simulink model "commhdlQPSKTxRxLoopback"  (R2025b)
settings: Solver=FixedStepDiscrete  StartTime=0.0  StopTime=stopTime  RelTol=1e-3
PostLoadFcn:
  | hScopeConfig = get_param([gcs '/Receiver/QPSK Rx/Frequency and Time Synchronizer/Symbol Synchronizer/No HDL/QPSK Receiver Eye Diagram'],'ScopeConfiguration');
  | 
  | hScopeConfig.OpenAtSimulationStart = false;
  | hScopeConfig.Visible = false;
  | SamplesPerSymbol = 4;
  | %UpsamplesRx = 1;
  | clear hScopeConfig
InitFcn:
  | commhdlQPSKTxRxModelInit;
  | % Rate bridge: ADRV9002/Jupiter radio runs at 15.36 MHz = 2x the 7.68 MHz
  | % (4 samples/symbol @ Rsym=1.92 MHz) the QPSK Rx requires. The deployed
  | % Receiver must downsample the ADC stream by 2. UpsamplesRx=1 fed the QPSK
  | % Rx 8 sps (2x-upsampled) and broke symbol sync / the loopback bit check.
  | UpsamplesRx = 1;   %% T8 RATE FIX: rail 15.36e6 == ADC bus rate,
  | %% no ingress decimation (was 2 when the rail sat on the 7.68e6 rung)
  | UpsamplesTx = 1;
  | clear simTimingOffset;
StopFcn:
  | if exist('simTimingOffset','var')
  |   disp('Simulation completed');
  |   %QPSKTxRxVerification;
  | end
undefined symbols (not defined in the file or in its folder): Add, Config, fsym, randsrc, RandStream, Rsym, Shift
libraries: hdlsllib x141, simulink x43, dspsigops x34, dsphdlfiltering2 x6, dsphdlsigops2 x4, dsphdlmathfun2 x4, commdigbbndpm3 x4, dspmlti4 x2, commchan3 x1, commrflib2 x1, commcnvcod2 x1
(part 6 of 8)

== system commhdlQPSKTxRxLoopback/TxRxComposite/Receiver/QPSK Rx/Frequency and Time Synchronizer/Preamble Detector/Peak Search ==
  note: peak picker
  corr : Inport
  thresholdExceeded : Inport  Port=2
  validIn : Inport  Port=3
  Compare To Constant : simulink/Logic and Bit Operations/Compare To Constant  relop===  const=samplesPerFrame1x - 1  OutDataTypeStr=boolean
  Logical Operator : Logic  IconShape=distinctive  AllPortsSameDT=off  OutDataTypeStr=boolean
  Logical Operator4 : Logic  IconShape=distinctive  AllPortsSameDT=off  OutDataTypeStr=boolean
  Relational Operator : RelationalOperator  Operator=>  OutDataTypeStr=boolean  InputSameDT=off
  Terminator : Terminator
  Unit Delay Enabled Synchronous : hdlsllib/Discrete/Unit Delay Enabled Synchronous  InitialCondition=0.0  SampleTime=-1
  Unit Delay Enabled Synchronous1 : hdlsllib/Discrete/Unit Delay Enabled Synchronous  InitialCondition=0.0  SampleTime=-1
  Unit Delay Enabled Resettable Synchronous : hdlsllib/Discrete/Unit Delay Enabled Resettable Synchronous  InitialCondition=0.0  SampleTime=-1
  Unit Delay Enabled Resettable Synchronous1 : hdlsllib/Discrete/Unit Delay Enabled Resettable Synchronous  InitialCondition=0.0  SampleTime=-1
  timing Reference : hdlsllib/Sources/HDL Counter  CountType=Count limited  CountInit=0  CountStep=1  CountMax=samplesPerFrame1x - 1  CountFromType=Initial value  CountFrom=0  CountResetPort=off  CountLoadPort=off  CountEnbPort=on  CountDirPort=off  CountHitOutputPort=off  CountDataType=Unsigned  CountWordLen=nextpow2(samplesPerFrame1x - 1)  CountFracLen=0  CountSampTime=1
  timing Reference Long : hdlsllib/Sources/HDL Counter  CountType=Free running  CountInit=0  CountStep=1  CountMax=samplesPerFrame1x - 1  CountFromType=Initial value  CountFrom=0  CountResetPort=off  CountLoadPort=off  CountEnbPort=on  CountDirPort=off  CountHitOutputPort=off  CountDataType=Unsigned  CountWordLen=32  CountFracLen=0  CountSampTime=1
  timingOffset : Outport
  done : Outport  Port=2
  success : Outport  Port=3
  p1c_tref : Outport  Port=4
  p1c_treflong : Outport  Port=5
  p1c_runmax : Outport  Port=6
  p1c_newpk : Outport  Port=7
  p1c_heldts : Outport  Port=8
  wires:
  Unit Delay Enabled Synchronous1/1 -> Terminator/1, p1c_heldts/1
  Unit Delay Enabled Synchronous/1 -> timingOffset/1
  Logical Operator4/1 -> Unit Delay Enabled Resettable Synchronous/2, Unit Delay Enabled Synchronous1/2, Unit Delay Enabled Synchronous/2, p1c_newpk/1
  Unit Delay Enabled Resettable Synchronous1/1 -> success/1
  Unit Delay Enabled Resettable Synchronous/1 -> Relational Operator/2, p1c_runmax/1
  Relational Operator/1 -> Logical Operator4/1
  Logical Operator/1 -> Unit Delay Enabled Resettable Synchronous/3, done/1, Unit Delay Enabled Resettable Synchronous1/3
  Compare To Constant/1 -> Logical Operator/2
  corr/1 -> Relational Operator/1, Unit Delay Enabled Resettable Synchronous/1
  thresholdExceeded/1 -> Logical Operator4/2, Unit Delay Enabled Resettable Synchronous1/1, Unit Delay Enabled Resettable Synchronous1/2
  timing Reference/1 -> Compare To Constant/1, Unit Delay Enabled Synchronous/1, p1c_tref/1
  timing Reference Long/1 -> Unit Delay Enabled Synchronous1/1, p1c_treflong/1
  validIn/1 -> timing Reference Long/1, timing Reference/1, Logical Operator/1

== system commhdlQPSKTxRxLoopback/TxRxComposite/Receiver/QPSK Rx/Frequency and Time Synchronizer/Preamble Detector/Timing Adjust ==
  timingOffset : Inport
  timingOffsetValid : Inport  Port=2
  dataIn : Inport  Port=3
  validIn : Inport  Port=4
  Delay{,1..4} (5 alike) : Delay  DelayLength=1
  Logical Operator : Logic  AllPortsSameDT=off  OutDataTypeStr=boolean
  Logical Operator1 : Logic  Operator=NOT  AllPortsSameDT=off  OutDataTypeStr=boolean
  Logical Operator2 : Logic  Inputs=3  AllPortsSameDT=off  OutDataTypeStr=boolean
  No HDL : Subsystem
  Relational Operator : RelationalOperator  Operator===  OutDataTypeStr=boolean  InputSameDT=off
  State Register : hdlsllib/Discrete/Unit Delay Enabled Resettable Synchronous  InitialCondition=0.0  SampleTime=-1
  Unit Delay Enabled Synchronous3 : hdlsllib/Discrete/Unit Delay Enabled Synchronous  InitialCondition=0.0  SampleTime=-1
  timing Reference : hdlsllib/Sources/HDL Counter  CountType=Count limited  CountInit=0  CountStep=1  CountMax=searchSamples - 1  CountFromType=Initial value  CountFrom=0  CountResetPort=off  CountLoadPort=off  CountEnbPort=on  CountDirPort=off  CountHitOutputPort=off  CountDataType=Unsigned  CountWordLen=nextpow2(searchSamples - 1)  CountFracLen=0  CountSampTime=1
  dataOut : Outport
  validOut : Outport  Port=2
  SyncPulse : Outport  Port=3
  p1c_armed : Outport  Port=4
  p1c_taref : Outport  Port=5
  p1c_accoff : Outport  Port=6
  wires:
  dataIn/1 -> Delay4/1
  Delay1/1 -> Logical Operator1/1
  timingOffsetValid/1 -> Logical Operator/1, Unit Delay Enabled Synchronous3/2, State Register/1, State Register/2
  timing Reference/1 -> Relational Operator/1, No HDL/2(timingOffset), p1c_taref/1
  Delay2/1 -> State Register/3
  Logical Operator2/1 -> Delay2/1, Delay/1, No HDL/3(syncPulse)
  Relational Operator/1 -> Logical Operator2/2
  Logical Operator1/1 -> Logical Operator/2
  State Register/1 -> Delay1/1, Logical Operator2/3, p1c_armed/1
  validIn/1 -> Delay3/1, No HDL/1(validIn), Logical Operator2/1, timing Reference/1
  Delay/1 -> SyncPulse/1
  Unit Delay Enabled Synchronous3/1 -> Relational Operator/2, p1c_accoff/1
  timingOffset/1 -> Unit Delay Enabled Synchronous3/1
  Delay3/1 -> validOut/1
  Delay4/1 -> dataOut/1

== system commhdlQPSKTxRxLoopback/TxRxComposite/Receiver/QPSK Rx/Frequency and Time Synchronizer/Symbol Synchronizer/Gardner TED ==
  data : Inport
  strobe : Inport  Port=2
  Constant : Constant  Value=0  OutDataTypeStr=Inherit: Inherit via back propagation  SampleTime=1/(Rsym*SamplesPerSymbol)
  Delay10 : Delay  DelayLength=4
  GTED : Subsystem
  Switch : Switch  Criteria=u2 ~= 0  InputSameDT=off
  e : Outport  VectorParamsAs1DForOutWhenUnconnected=off
  wires:
  Delay10/1 -> Switch/2
  GTED/1(Out1) -> Switch/1
  data/1 -> GTED/1(In1)
  strobe/1 -> Delay10/1
  Switch/1 -> e/1
  Constant/1 -> Switch/3

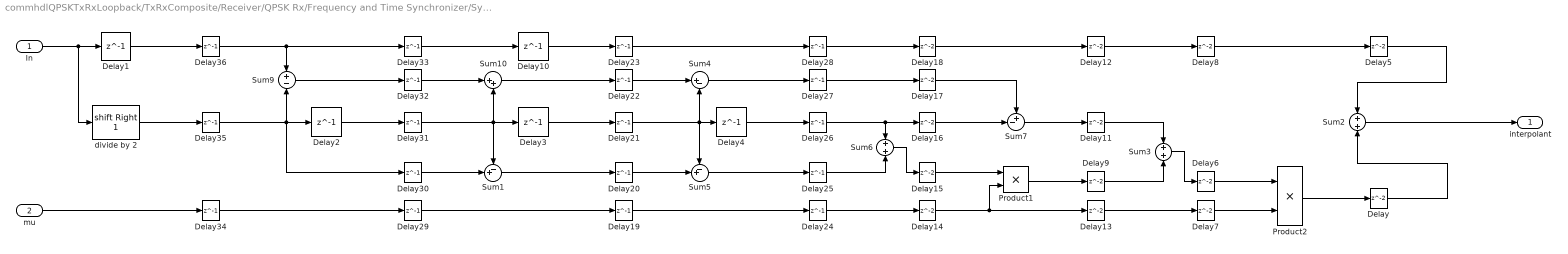
== system commhdlQPSKTxRxLoopback/TxRxComposite/Receiver/QPSK Rx/Frequency and Time Synchronizer/Symbol Synchronizer/Interpolation Filter ==
  In : Inport
  mu : Inport  Port=2
  Delay{,5..9,11..18} (14 alike) : Delay
  Delay{1..4,10} (5 alike) : Delay  DelayLength=1  InitialCondition=0
  Delay{19..36} (18 alike) : Delay  DelayLength=1
  Product1 : Product  OutDataTypeStr=fixdt(1,16,10)  RndMeth=Zero
  Product2 : Product  RndMeth=Zero  OutDataTypeStr=Inherit: Same as first input
  Sum1 : Sum  Inputs=-+|
  Sum10 : Sum  Inputs=|++
  Sum2 : Sum  Inputs=+|+
  Sum3 : Sum  Inputs=+|+  OutDataTypeStr=fixdt(1,16,10)
  Sum4 : Sum  Inputs=|+-
  Sum5 : Sum  Inputs=-+|
  Sum6 : Sum  Inputs=+|+  OutDataTypeStr=fixdt(1,16,11)  SaturateOnIntegerOverflow=on
  Sum7 : Sum  Inputs=+-|  OutDataTypeStr=fixdt(1,16,10)
  Sum9 : Sum  Inputs=+-
  divide by 2 : ArithShift  BitShiftNumber=1  BitShiftDirection=Right
  interpolant : Outport
  wires:
  Delay36/1 -> Sum9/1, Delay33/1
  Delay35/1 -> Sum9/2, Delay2/1, Delay30/1
  Delay34/1 -> Delay29/1
  Delay33/1 -> Delay10/1
  Delay32/1 -> Sum10/1
  Delay31/1 -> Delay3/1, Sum10/2, Sum1/1
  Delay30/1 -> Sum1/2
  Delay29/1 -> Delay19/1
  Delay23/1 -> Delay28/1
  Delay22/1 -> Sum4/1
  Delay21/1 -> Delay4/1, Sum5/1, Sum4/2
  Delay20/1 -> Sum5/2
  Delay19/1 -> Delay24/1
  Delay25/1 -> Sum6/2
  Delay28/1 -> Delay18/1
  Delay27/1 -> Delay17/1
  Delay26/1 -> Sum6/1, Delay16/1
  Sum6/1 -> Delay15/1
  Delay24/1 -> Delay14/1
  Delay10/1 -> Delay23/1
  Sum4/1 -> Delay27/1
  Delay4/1 -> Delay26/1
  Sum5/1 -> Delay25/1
  mu/1 -> Delay34/1
  Delay18/1 -> Delay12/1
  Delay17/1 -> Sum7/1
  Delay16/1 -> Sum7/2
  Delay15/1 -> Product1/1
  Delay14/1 -> Product1/2, Delay13/1
  Delay13/1 -> Delay7/1
  Delay12/1 -> Delay8/1
  Delay11/1 -> Sum3/1
  Delay9/1 -> Sum3/2
  Delay8/1 -> Delay5/1
  Delay7/1 -> Product2/2
  Delay6/1 -> Product2/1
  Delay5/1 -> Sum2/1
  Delay/1 -> Sum2/2
  divide by 2/1 -> Delay35/1
  Delay1/1 -> Delay36/1
  Delay2/1 -> Delay31/1
  Sum10/1 -> Delay22/1
  Delay3/1 -> Delay21/1
  Sum1/1 -> Delay20/1
  Sum3/1 -> Delay6/1
  Product2/1 -> Delay/1
  Product1/1 -> Delay9/1
  Sum7/1 -> Delay11/1
  Sum2/1 -> interpolant/1
  In/1 -> Delay1/1, divide by 2/1
  Sum9/1 -> Delay32/1

== system commhdlQPSKTxRxLoopback/TxRxComposite/Receiver/QPSK Rx/Frequency and Time Synchronizer/Symbol Synchronizer/Loop Filter ==
  note: Proportional-Plus-Integrator Loop Filter,
      | Infinite DC Response to guarantee convergence
  e : Inport
  ss_prop_gain : Inport  Port=2  OutDataTypeStr=uint32  SampleTime=1/(Rsym*SamplesPerSymbol)
  ss_integ_gain : Inport  Port=3  OutDataTypeStr=uint32  SampleTime=1/(Rsym*SamplesPerSymbol)
  Add : Sum
  Add2 : Sum  Inputs=|++  OutDataTypeStr=Inherit: Same as first input
  Data Type Conversion17 : DataTypeConversion  OutDataTypeStr=fixdt(1,11,10)  RndMeth=Floor
  Delay : Delay  DelayLength=1
  Delay1 : Delay  DelayLength=1  InitialCondition=0
  Delay2 : Delay  InitialCondition=0
  Delay3 : Delay  InitialCondition=0
  Delay4 : Delay  DelayLength=1  InitialCondition=0
  Delay5 : Delay  InitialCondition=0
  Delay6 : Delay  DelayLength=1
  IntegClamp : Saturate  UpperLimit=0.06  LowerLimit=-0.06
  K1 : Gain  Gain=fi(SSLoopFilterPropGain,1,24,24)  ParamDataTypeStr=Inherit: Inherit from 'Gain'  OutDataTypeStr=fixdt(1,30,23)
  K2 : Gain  Gain=fi(SSLoopFilterIntegGain,1,24,24)  ParamDataTypeStr=Inherit: Inherit from 'Gain'  OutDataTypeStr=fixdt(1,30,23)
  LGMux_ss_integ_gain : MATLAB Function  TreatAsAtomicUnit=on
  LGMux_ss_prop_gain : MATLAB Function  TreatAsAtomicUnit=on
  LGProd_ss_integ_gain : Product  OutDataTypeStr=fixdt(1,30,23)
  LGProd_ss_prop_gain : Product  OutDataTypeStr=fixdt(1,30,23)
  LGSw_ss_integ_gain : Switch  Criteria=u2 ~= 0  OutDataTypeStr=fixdt(1,30,23)
  LGSw_ss_prop_gain : Switch  Criteria=u2 ~= 0  OutDataTypeStr=fixdt(1,30,23)
  v : Outport
  wires:
  IntegClamp/1 -> Delay4/1, Delay/1
  Add2/1 -> IntegClamp/1
  Delay6/1 -> Add2/1
  Data Type Conversion17/1 -> v/1
  Delay2/1 -> K2/1, K1/1, LGProd_ss_prop_gain/1, LGProd_ss_integ_gain/1
  Delay4/1 -> Add/2
  Delay1/1 -> Add/1
  Add/1 -> Data Type Conversion17/1
  e/1 -> Delay2/1
  Delay3/1 -> Delay1/1
  Delay5/1 -> Delay6/1
  Delay/1 -> Add2/2
  ss_prop_gain/1 -> LGMux_ss_prop_gain/1(axi)
  LGMux_ss_prop_gain/1(coeff) -> LGProd_ss_prop_gain/2
  LGProd_ss_prop_gain/1 -> LGSw_ss_prop_gain/1
  LGMux_ss_prop_gain/2(nz) -> LGSw_ss_prop_gain/2
  K1/1 -> LGSw_ss_prop_gain/3
  LGSw_ss_prop_gain/1 -> Delay3/1
  ss_integ_gain/1 -> LGMux_ss_integ_gain/1(axi)
  LGMux_ss_integ_gain/1(coeff) -> LGProd_ss_integ_gain/2
  LGProd_ss_integ_gain/1 -> LGSw_ss_integ_gain/1
  LGMux_ss_integ_gain/2(nz) -> LGSw_ss_integ_gain/2
  K2/1 -> LGSw_ss_integ_gain/3
  LGSw_ss_integ_gain/1 -> Delay5/1

== system commhdlQPSKTxRxLoopback/TxRxComposite/Receiver/QPSK Rx/Frequency and Time Synchronizer/Symbol Synchronizer/No HDL ==
  data : Inport
  valid : Inport  Port=2
  Data Type Conversion : DataTypeConversion  OutDataTypeStr=double  SaturateOnIntegerOverflow=off  RndMeth=Floor
  No HDL : Subsystem
  QPSK Receiver Eye Diagram : EyeDiagramBlock  WindowPosition=[403.000000,370.000000,417.000000,506.000000,]  ScopeFrameLocation=window  SamplesPerSymbol=SamplesPerSymbol  SymbolsPerTrace=1  Title=RRC Matched Filtered Output  YLimits=[-1.1602,1.2629]
      settings: OpenAtSimulationStart=off
  Unit Delay Enabled Synchronous : hdlsllib/Discrete/Unit Delay Enabled Synchronous  InitialCondition=0.0  SampleTime=-1
  wires:
  Data Type Conversion/1 -> QPSK Receiver Eye Diagram/1
  valid/1 -> No HDL/Enable, Unit Delay Enabled Synchronous/2
  Unit Delay Enabled Synchronous/1 -> Data Type Conversion/1
  data/1 -> Unit Delay Enabled Synchronous/1, No HDL/1(data)

== system commhdlQPSKTxRxLoopback/TxRxComposite/Receiver/QPSK Rx/Frequency and Time Synchronizer/Symbol Synchronizer/Rate Handle ==
  dataIn : Inport
  strobe : Inport  Port=2
  validIn : Inport  Port=3
  Compare To Constant : simulink/Logic and Bit Operations/Compare To Constant  relop===  const=0  OutDataTypeStr=boolean
  Constant : Constant  Value=false  SampleTime=-1
  FIFO : Subsystem  mask{fifoSize=32, pushFullDiag=Error, popEmptyDiag=Ignore}
      mask prompts: fifoSize "FIFO size:"; pushFullDiag "Push full FIFO:"; popEmptyDiag "Pop empty FIFO:"
      mask TypeOptions pushFullDiag: Ignore | Warning | Error
      mask TypeOptions popEmptyDiag: Ignore | Warning | Error
  HDL Counter : hdlsllib/Sources/HDL Counter  CountType=Count limited  CountInit=0  CountStep=1  CountMax=SamplesPerSymbol - 1  CountFromType=Initial value  CountFrom=0  CountResetPort=off  CountLoadPort=off  CountEnbPort=on  CountDirPort=off  CountHitOutputPort=off  CountDataType=Unsigned  CountWordLen=nextpow2(SamplesPerSymbol - 1)  CountFracLen=0  CountSampTime=1
  Logical Operator : Logic  AllPortsSameDT=off  OutDataTypeStr=boolean
  Terminator : Terminator
  dataOut : Outport
  validOut : Outport  Port=2
  wires:
  Constant/1 -> FIFO/4(reset)
  FIFO/2(numEntries) -> Terminator/1
  FIFO/3(validPop) -> validOut/1
  FIFO/1(out) -> dataOut/1
  Logical Operator/1 -> FIFO/3(pop)
  Compare To Constant/1 -> Logical Operator/2
  HDL Counter/1 -> Compare To Constant/1
  validIn/1 -> HDL Counter/1, Logical Operator/1
  dataIn/1 -> FIFO/1(in)
  strobe/1 -> FIFO/2(push)

== system commhdlQPSKTxRxLoopback/TxRxComposite/Transmitter/QPSK Tx/Bit Packetizer/Data Bits FIFO/No HDL ==
  push : Inport
  pop : Inport  Port=2
  MATLAB Function : MATLAB Function  TreatAsAtomicUnit=on
  No HDL : Subsystem
  wires:
  MATLAB Function/3(empty) -> No HDL/4(empty)
  MATLAB Function/1(full) -> No HDL/2(full)
  MATLAB Function/2(ncount) -> No HDL/3(ncount)
  pop/1 -> No HDL/5(pop), MATLAB Function/2(rd)
  push/1 -> No HDL/1(push), MATLAB Function/1(wr)

== system commhdlQPSKTxRxLoopback/TxRxComposite/Transmitter/QPSK Tx/Bit Packetizer/Preamble Bits Generator/Preamble Bits Store ==
  note: The Preamble is padded with zeros in the LUT such that
      | the length is the 2^nextpow2(length(Preamble)) for
      | efficient resource mapping to RAM
  actualPreamble : Inport
  sampleCount : Inport  Port=2
  Constant : Constant  OutDataTypeStr=boolean  SampleTime=1/(Rsym*SamplesPerSymbol)
  Extract Bits : simulink/Logic and Bit Operations/Extract Bits  bitsToExtract=Range of bits  numBits=8  bitIdxRange=[0 nextpow2(length(Preamble))-1]  outScalingMode=Treat bit field as an integer
  Preamble : LookupNDDirect  NumberOfTableDimensions=1  Table=[Preamble;false(32-length(Preamble),1)]  DiagnosticForOutOfRangeInput=Error
  Switch : Switch  Criteria=u2 ~= 0  Threshold=1  SaturateOnIntegerOverflow=off  InputSameDT=off
  preamble : Outport
  wires:
  actualPreamble/1 -> Switch/2
  sampleCount/1 -> Extract Bits/1
  Preamble/1 -> Switch/1
  Extract Bits/1 -> Preamble/1
  Constant/1 -> Switch/3
  Switch/1 -> preamble/1

== system commhdlQPSKTxRxLoopback/Receiver/QPSK Rx/Frequency and Time Synchronizer/Coarse Frequency Compensator/Coarse Frequency Estimator/Integrator/Reset Generator ==
  validIn : Inport
  Compare To Constant : simulink/Logic and Bit Operations/Compare To Constant  relop===  const=integAvgLen  OutDataTypeStr=boolean
  Delay1 : Delay  DelayLength=1
  Delay5 : Delay  DelayLength=1
  HDL Counter : hdlsllib/Sources/HDL Counter  CountType=Count limited  CountInit=0  CountStep=1  CountMax=integAvgLen  CountFromType=Initial value  CountFrom=0  CountResetPort=off  CountLoadPort=off  CountEnbPort=on  CountDirPort=off  CountHitOutputPort=off  CountDataType=Unsigned  CountWordLen=nextpow2(integAvgLen + 1)  CountFracLen=0  CountSampTime=1
  Logical Operator : Logic  AllPortsSameDT=off  OutDataTypeStr=boolean
  reset : Outport
  wires:
  Delay1/1 -> Logical Operator/1
  Delay5/1 -> Compare To Constant/1
  Logical Operator/1 -> reset/1
  validIn/1 -> HDL Counter/1, Delay1/1
  Compare To Constant/1 -> Logical Operator/2
  HDL Counter/1 -> Delay5/1

== system commhdlQPSKTxRxLoopback/Receiver/QPSK Rx/Frequency and Time Synchronizer/Phase Ambiguity Estimation and Correction/Phase Ambiguity Corrector/Reciprocal/Function Impl ==
  switch : Inport
  LUTAddr : Inport  Port=2
  Delay{6..8,10,15..16} (6 alike) : Delay
  Delay9 : Delay  DelayLength=1
  LUT1 : LookupNDDirect  NumberOfTableDimensions=1  Table=LUT(:,1)  DiagnosticForOutOfRangeInput=Error
  LUT2 : LookupNDDirect  NumberOfTableDimensions=1  Table=LUT(:,2)  DiagnosticForOutOfRangeInput=Error
  Multiport Switch : MultiPortSwitch  DataPortOrder=Zero-based contiguous  Inputs=2  zeroidx=on  SaturateOnIntegerOverflow=off  InputSameDT=off
  functionValues : Outport
  wires:
  Multiport Switch/1 -> Delay9/1
  Delay6/1 -> LUT1/1
  Delay7/1 -> LUT2/1
  Delay8/1 -> Delay10/1
  switch/1 -> Delay8/1
  LUT1/1 -> Delay16/1
  LUT2/1 -> Delay15/1
  Delay9/1 -> functionValues/1
  Delay10/1 -> Multiport Switch/1
  Delay16/1 -> Multiport Switch/3
  Delay15/1 -> Multiport Switch/2
  LUTAddr/1 -> Delay6/1, Delay7/1

== system commhdlQPSKTxRxLoopback/Receiver/QPSK Rx/Frequency and Time Synchronizer/Preamble Detector/FIFO/Validate Input Push Pop/No HDL ==
  pushFullFIFO : Inport
  popEmptyFIFO : Inport  Port=2
  Constant2 : Constant  Value=pushFullDiag  SampleTime=-1
  Constant3 : Constant  Value=popEmptyDiag  SampleTime=-1
  MATLAB Function : MATLAB Function  TreatAsAtomicUnit=on
  wires:
  Constant2/1 -> MATLAB Function/1(pushFullDiag)
  Constant3/1 -> MATLAB Function/2(popEmptyDiag)
  popEmptyFIFO/1 -> MATLAB Function/4(popEmpty)
  pushFullFIFO/1 -> MATLAB Function/3(pushFull)

== system commhdlQPSKTxRxLoopback/Receiver/QPSK Rx/Frequency and Time Synchronizer/Preamble Detector/Timing Adjust/No HDL/No HDL ==
  timingOffset : Inport
  Enable : EnablePort
  Data Type Conversion : DataTypeConversion  OutDataTypeStr=double  SaturateOnIntegerOverflow=off  RndMeth=Floor
  To Workspace : ToWorkspace  VariableName=simTimingOffset  SampleTime=-1
      settings: Save2DSignal=2-D array (concatenate along first dimension)
  wires:
  Data Type Conversion/1 -> To Workspace/1
  timingOffset/1 -> Data Type Conversion/1

== system commhdlQPSKTxRxLoopback/Receiver/QPSK Rx/Frequency and Time Synchronizer/Preamble Detector/Timing Adjust/No HDL/No HDL1 ==
  frameNumber : Inport
  Enable : EnablePort
  Data Type Conversion : DataTypeConversion  OutDataTypeStr=double  SaturateOnIntegerOverflow=off  RndMeth=Floor
  To Workspace : ToWorkspace  VariableName=simSyncedPackets  SampleTime=-1
      settings: Save2DSignal=2-D array (concatenate along first dimension)
  wires:
  frameNumber/1 -> Data Type Conversion/1
  Data Type Conversion/1 -> To Workspace/1

== system commhdlQPSKTxRxLoopback/Receiver/QPSK Rx/Frequency and Time Synchronizer/Symbol Synchronizer/Rate Handle/FIFO/Validate Input Push Pop ==
  rst : Inport
  push : Inport  Port=2
  pop : Inport  Port=3
  Compare To Constant : hdlsllib/Logic and Bit Operations/Compare To Constant  relop===  const=0  OutDataTypeStr=boolean
  Compare To Constant1 : hdlsllib/Logic and Bit Operations/Compare To Constant  relop===  const=fifoSize  OutDataTypeStr=boolean
  Constant : Constant  Value=true  SampleTime=-1
  Constant1 : Constant  Value=false  SampleTime=-1
  Delay : Delay  DelayLength=1
  Logical Operator1 : Logic  Operator=XOR  AllPortsSameDT=off  OutDataTypeStr=boolean
  Logical Operator2 : Logic  Operator=NOT  AllPortsSameDT=off  OutDataTypeStr=boolean
  Logical Operator{3..5,7,9} (5 alike) : Logic  AllPortsSameDT=off  OutDataTypeStr=boolean
  Logical Operator6 : Logic  Operator=NOT  AllPortsSameDT=off  OutDataTypeStr=boolean
  Logical Operator8 : Logic  Operator=NOT  AllPortsSameDT=off  OutDataTypeStr=boolean
  MATLAB Function : MATLAB Function  TreatAsAtomicUnit=on  mask{initVal=0, countToVal=fifoSize}
      mask prompts: initVal "Initial value:"; countToVal "Count to value:"
  No HDL : Subsystem
  Switch : Switch  Criteria=u2 ~= 0  SaturateOnIntegerOverflow=off  InputSameDT=off
  valid push : Outport
  valid pop : Outport  Port=2
  numEntries : Outport  Port=3
  wires:
  Logical Operator9/1 -> Logical Operator1/1, valid push/1
  Logical Operator2/1 -> Logical Operator9/2
  Logical Operator5/1 -> Logical Operator4/1
  Logical Operator8/1 -> Logical Operator5/2
  push/1 -> Logical Operator5/1, Logical Operator9/1
  Logical Operator1/1 -> MATLAB Function/2(enb)
  Logical Operator6/1 -> Logical Operator7/2
  Logical Operator7/1 -> Switch/2, valid pop/1, Logical Operator8/1, Logical Operator1/2
  Compare To Constant1/1 -> Logical Operator4/2
  Constant/1 -> Switch/3
  Logical Operator4/1 -> No HDL/1(pushFullFIFO), Logical Operator2/1  "push on full FIFO"
  Logical Operator3/1 -> No HDL/2(popEmptyFIFO), Logical Operator6/1  "pop on empty FIFO"
  Constant1/1 -> Switch/1
  MATLAB Function/1(count) -> Delay/1
  Switch/1 -> MATLAB Function/3(dir)
  pop/1 -> Logical Operator3/2, Logical Operator7/1
  Compare To Constant/1 -> Logical Operator3/1
  rst/1 -> MATLAB Function/1(rst)
  Delay/1 -> Compare To Constant1/1, numEntries/1, Compare To Constant/1

== system commhdlQPSKTxRxLoopback/TxRxComposite/Receiver/QPSK Rx/Frequency and Time Synchronizer/Coarse Frequency Compensator/Coarse Frequency Estimator/Extract Frequency ==
  datain : Inport
  validIn : Inport  Port=2
  Complex to Magnitude-Angle HDL Optimized : dsphdlmathfun2/Complex to Magnitude-Angle  NumIterationsSource=Auto  NumIterations=10  OutputFormat=Angle  AngleFormat=Normalized  ScaleOutput=on  ScalingMethod=Shift-Add  SimulateUsing=Code generation
  Delay{1..4} (4 alike) : Delay  DelayLength=1
  Gain : Gain  Gain=1/2  ParamDataTypeStr=fixdt(0,1,1)  OutDataTypeStr=Inherit: Same as input
  Unit Delay Enabled Synchronous : hdlsllib/Discrete/Unit Delay Enabled Synchronous  InitialCondition=0.0  SampleTime=-1
  normFreqOut : Outport
  wires:
  Complex to Magnitude-Angle HDL Optimized/1 -> Unit Delay Enabled Synchronous/1
  Delay4/1 -> Complex to Magnitude-Angle HDL Optimized/2
  validIn/1 -> Delay4/1
  Delay3/1 -> normFreqOut/1
  Delay2/1 -> Gain/1
  Delay1/1 -> Complex to Magnitude-Angle HDL Optimized/1
  Gain/1 -> Delay3/1
  datain/1 -> Delay1/1
  Complex to Magnitude-Angle HDL Optimized/2 -> Unit Delay Enabled Synchronous/2
  Unit Delay Enabled Synchronous/1 -> Delay2/1

== system commhdlQPSKTxRxLoopback/TxRxComposite/Receiver/QPSK Rx/Frequency and Time Synchronizer/Coarse Frequency Compensator/Coarse Frequency Estimator/Integrator ==
  note: store the value in the Reg before reset
  dataIn : Inport
  validIn : Inport  Port=2
  Add1 : Sum  Inputs=|++  OutDataTypeStr=Inherit: Same as first input
  Delay : Delay  DelayLength=1
  Delay1 : Delay  DelayLength=1
  Delay2 : Delay  DelayLength=1
  Integ Reg : hdlsllib/Discrete/Unit Delay Enabled Resettable Synchronous  InitialCondition=0.0  SampleTime=-1
  Reset Generator : Subsystem
  Store Reg : hdlsllib/Discrete/Unit Delay Enabled Synchronous  InitialCondition=0.0  SampleTime=-1
  IntegOut : Outport
  IntegValid : Outport  Port=2
  wires:
  Delay2/1 -> Integ Reg/2
  Reset Generator/1(reset) -> Integ Reg/3, Store Reg/2, Delay/1
  Store Reg/1 -> IntegOut/1
  Delay/1 -> IntegValid/1
  Delay1/1 -> Add1/1
  dataIn/1 -> Delay1/1
  validIn/1 -> Reset Generator/1(validIn), Delay2/1
  Integ Reg/1 -> Add1/2, Store Reg/1
  Add1/1 -> Integ Reg/1

== system commhdlQPSKTxRxLoopback/TxRxComposite/Receiver/QPSK Rx/Frequency and Time Synchronizer/Phase Ambiguity Estimation and Correction/Phase Ambiguity Corrector/Reciprocal ==
  dataIn : Inport
  Compare To Constant : simulink/Logic and Bit Operations/Compare To Constant  relop=<  const=0  OutDataTypeStr=boolean
  Data Type Conversion : DataTypeConversion  OutDataTypeStr=fixdt(1,WL,0)  ConvertRealWorld=Stored Integer (SI)  SaturateOnIntegerOverflow=off  RndMeth=Floor
  Data Type Conversion1 : DataTypeConversion  OutDataTypeStr=fixdt(0,LUTAddrWL,0)  ConvertRealWorld=Stored Integer (SI)  SaturateOnIntegerOverflow=off  RndMeth=Floor
  Data Type Conversion2 : DataTypeConversion  OutDataTypeStr=fixdt(0,WL-LUTAddrWL,0)  ConvertRealWorld=Stored Integer (SI)  SaturateOnIntegerOverflow=off  RndMeth=Floor
  Delay : Delay  DelayLength=1
  Delay1 : Delay  DelayLength=1
  Delay2 : Delay  DelayLength=1
  Extract Bits : simulink/Logic and Bit Operations/Extract Bits  bitsToExtract=Range ending with least significant bit  numBits=LUTAddrWL  bitIdxRange=[0 7]  outScalingMode=Treat bit field as an integer
  Function Impl : Subsystem
  dataOut : Outport
  wires:
  Data Type Conversion2/1 -> Function Impl/1(switch)
  Delay2/1 -> Data Type Conversion1/1
  Delay1/1 -> Data Type Conversion2/1
  Delay/1 -> Extract Bits/1, Compare To Constant/1
  Function Impl/1(functionValues) -> dataOut/1
  Data Type Conversion1/1 -> Function Impl/2(LUTAddr)
  Compare To Constant/1 -> Delay1/1
  Data Type Conversion/1 -> Delay/1
  Extract Bits/1 -> Delay2/1
  dataIn/1 -> Data Type Conversion/1

== system commhdlQPSKTxRxLoopback/TxRxComposite/Receiver/QPSK Rx/Frequency and Time Synchronizer/Phase Ambiguity Estimation and Correction/Phase Ambiguity Estimator/Subsystem ==
  L : Inport
  H : Inport  Port=2
  Delay6 : Delay  DelayLength=1  InitialCondition=1
  Logical Operator : Logic  AllPortsSameDT=off  OutDataTypeStr=boolean
  Logical Operator1 : Logic  Operator=NOT  IconShape=distinctive  AllPortsSameDT=off  OutDataTypeStr=boolean
  Logical Operator2 : Logic  Operator=OR  AllPortsSameDT=off  OutDataTypeStr=boolean
  Out2 : Outport
  wires:
  Logical Operator2/1 -> Delay6/1
  Logical Operator/1 -> Logical Operator2/2
  Logical Operator1/1 -> Logical Operator/1
  Delay6/1 -> Logical Operator/2, Out2/1
  H/1 -> Logical Operator2/1
  L/1 -> Logical Operator1/1

== system commhdlQPSKTxRxLoopback/TxRxComposite/Receiver/QPSK Rx/Frequency and Time Synchronizer/Phase Ambiguity Estimation and Correction/Phase Ambiguity Estimator/Subsystem1 ==
  In1 : Inport
  validIn : Inport  Port=2
  Logical Operator1 : Logic  IconShape=distinctive  AllPortsSameDT=off  OutDataTypeStr=boolean
  Logical Operator2 : Logic  Operator=NOT  IconShape=distinctive  AllPortsSameDT=off  OutDataTypeStr=boolean
  validOut : Outport
  wires:
  Logical Operator2/1 -> Logical Operator1/1
  Logical Operator1/1 -> validOut/1
  validIn/1 -> Logical Operator1/2
  In1/1 -> Logical Operator2/1

== system commhdlQPSKTxRxLoopback/TxRxComposite/Receiver/QPSK Rx/Frequency and Time Synchronizer/Preamble Detector/Correlator/Magnitude Squared ==
  In1 : Inport
  Delay1 : Delay
  Delay2 : Delay
  Delay3 : Delay
  Math Function : Math  Operator=conj
  Product : Product
  Out1 : Outport
  wires:
  Delay3/1 -> Out1/1
  Delay1/1 -> Product/2
  Delay2/1 -> Product/1
  Product/1 -> Delay3/1
  Math Function/1 -> Delay1/1
  In1/1 -> Delay2/1, Math Function/1

== system commhdlQPSKTxRxLoopback/TxRxComposite/Receiver/QPSK Rx/Frequency and Time Synchronizer/Preamble Detector/Correlator/Magnitude Squared and Moving Sum ==
  scaled1 : Inport
  validIn : Inport  Port=2
  Add : Sum  Inputs=|+-  OutDataTypeStr=Inherit: Same as first input
  Add1 : Sum  Inputs=|++  OutDataTypeStr=Inherit: Same as first input
  Complex to Real-Imag1 : ComplexToRealImag  Output=Real
  Delay : Delay  DelayLength=13  ShowEnablePort=on
      settings: InputPortMap=u0,e6
  Delay{1..4,6,8..10,12} (9 alike) : Delay
  Delay11 : Delay  DelayLength=11
  Delay14 : Delay  DelayLength=1  ShowEnablePort=on
      settings: InputPortMap=u0,e6
  Delay5 : Delay  DelayLength=1
  Delay7 : Delay  DelayLength=1
  Gain : Gain  Gain=ThresoldGainFac  OutDataTypeStr=Inherit: Same as input
  Math Function1 : Math  Operator=conj
  Product1 : Product
  E1 : Outport
  wires:
  Delay12/1 -> Delay10/1
  Delay10/1 -> Delay9/1
  Delay9/1 -> Delay8/1
  Delay8/1 -> Delay7/1, Delay/2
  Delay7/1 -> Delay14/2
  Delay5/1 -> Add1/1
  Delay4/1 -> Add/1, Delay/1
  Delay3/1 -> Gain/1
  Delay2/1 -> Complex to Real-Imag1/1
  Delay1/1 -> Product1/2
  Delay6/1 -> Product1/1
  Gain/1 -> Delay4/1
  Product1/1 -> Delay2/1
  Math Function1/1 -> Delay1/1
  scaled1/1 -> Math Function1/1, Delay6/1
  Delay11/1 -> E1/1
  Add1/1 -> Delay14/1, Delay11/1
  Complex to Real-Imag1/1 -> Delay3/1
  Delay14/1 -> Add1/2
  Delay/1 -> Add/2
  validIn/1 -> Delay12/1
  Add/1 -> Delay5/1

== system commhdlQPSKTxRxLoopback/TxRxComposite/Receiver/QPSK Rx/Frequency and Time Synchronizer/Preamble Detector/FIFO/Validate Input Push Pop ==
  rst : Inport
  push : Inport  Port=2
  pop : Inport  Port=3
  Compare To Constant : hdlsllib/Logic and Bit Operations/Compare To Constant  relop===  const=0  OutDataTypeStr=boolean
  Compare To Constant1 : hdlsllib/Logic and Bit Operations/Compare To Constant  relop===  const=fifoSize  OutDataTypeStr=boolean
  Constant : Constant  Value=true  SampleTime=-1
  Constant1 : Constant  Value=false  SampleTime=-1
  Delay : Delay  DelayLength=1
  Logical Operator1 : Logic  Operator=XOR  AllPortsSameDT=off  OutDataTypeStr=boolean
  Logical Operator2 : Logic  Operator=NOT  AllPortsSameDT=off  OutDataTypeStr=boolean
  Logical Operator{3..5,7,9} (5 alike) : Logic  AllPortsSameDT=off  OutDataTypeStr=boolean
  Logical Operator6 : Logic  Operator=NOT  AllPortsSameDT=off  OutDataTypeStr=boolean
  Logical Operator8 : Logic  Operator=NOT  AllPortsSameDT=off  OutDataTypeStr=boolean
  MATLAB Function : MATLAB Function  TreatAsAtomicUnit=on  mask{initVal=0, countToVal=fifoSize}
      mask prompts: initVal "Initial value:"; countToVal "Count to value:"
  No HDL : Subsystem
  Switch : Switch  Criteria=u2 ~= 0  SaturateOnIntegerOverflow=off  InputSameDT=off
  valid push : Outport
  valid pop : Outport  Port=2
  numEntries : Outport  Port=3
  wires:
  Delay/1 -> Compare To Constant/1, numEntries/1, Compare To Constant1/1
  rst/1 -> MATLAB Function/1(rst)
  Compare To Constant/1 -> Logical Operator3/1
  pop/1 -> Logical Operator7/1, Logical Operator3/2
  Switch/1 -> MATLAB Function/3(dir)
  MATLAB Function/1(count) -> Delay/1
  Constant1/1 -> Switch/1
  Logical Operator3/1 -> Logical Operator6/1, No HDL/2(popEmptyFIFO)  "pop on empty FIFO"
  Logical Operator4/1 -> Logical Operator2/1, No HDL/1(pushFullFIFO)  "push on full FIFO"
  Constant/1 -> Switch/3
  Compare To Constant1/1 -> Logical Operator4/2
  Logical Operator7/1 -> Logical Operator1/2, Logical Operator8/1, valid pop/1, Switch/2
  Logical Operator6/1 -> Logical Operator7/2
  Logical Operator1/1 -> MATLAB Function/2(enb)
  push/1 -> Logical Operator9/1, Logical Operator5/1
  Logical Operator8/1 -> Logical Operator5/2
  Logical Operator5/1 -> Logical Operator4/1
  Logical Operator2/1 -> Logical Operator9/2
  Logical Operator9/1 -> valid push/1, Logical Operator1/1

== system commhdlQPSKTxRxLoopback/TxRxComposite/Receiver/QPSK Rx/Frequency and Time Synchronizer/Preamble Detector/Timing Adjust/No HDL ==
  note: This subsystem generates variables required for QPSKRxVerification for validation
  validIn : Inport
  timingOffset : Inport  Port=2
  syncPulse : Inport  Port=3
  Compare To Constant : simulink/Logic and Bit Operations/Compare To Constant  relop===  const=0  OutDataTypeStr=boolean
  Delay : Delay  DelayLength=4
  Delay1 : Delay  DelayLength=4
  Frame Counter : hdlsllib/Sources/HDL Counter  CountType=Free running  CountInit=0  CountStep=1  CountMax=bitsPerPacket/2 - 1  CountFromType=Initial value  CountFrom=0  CountResetPort=off  CountLoadPort=off  CountEnbPort=on  CountDirPort=off  CountHitOutputPort=off  CountDataType=Unsigned  CountWordLen=32  CountFracLen=0  CountSampTime=1
  Logical Operator : Logic  AllPortsSameDT=off  OutDataTypeStr=boolean
  No HDL : Subsystem
  No HDL1 : Subsystem
  Symbol Counter : hdlsllib/Sources/HDL Counter  CountType=Count limited  CountInit=0  CountStep=1  CountMax=bitsPerPacket/2 - 1  CountFromType=Initial value  CountFrom=0  CountResetPort=off  CountLoadPort=off  CountEnbPort=on  CountDirPort=off  CountHitOutputPort=off  CountDataType=Unsigned  CountWordLen=nextpow2(bitsPerPacket/2 - 1)  CountFracLen=0  CountSampTime=1
  Unit Delay Enabled Synchronous : hdlsllib/Discrete/Unit Delay Enabled Synchronous  InitialCondition=0.0  SampleTime=-1
  wires:
  Delay1/1 -> No HDL/1(timingOffset)
  Delay/1 -> No HDL1/Enable, No HDL/Enable
  Unit Delay Enabled Synchronous/1 -> No HDL1/1(frameNumber)
  syncPulse/1 -> Delay/1
  Frame Counter/1 -> Unit Delay Enabled Synchronous/1
  Compare To Constant/1 -> Logical Operator/1
  Logical Operator/1 -> Frame Counter/1, Unit Delay Enabled Synchronous/2
  Symbol Counter/1 -> Compare To Constant/1
  validIn/1 -> Symbol Counter/1, Logical Operator/2
  timingOffset/1 -> Delay1/1

== system commhdlQPSKTxRxLoopback/TxRxComposite/Receiver/QPSK Rx/Frequency and Time Synchronizer/Symbol Synchronizer/Gardner TED/GTED ==
  In1 : Inport
  Add : Sum
  Add1 : Sum  Inputs=+-
  Add2 : Sum  Inputs=+-
  Complex to Real-Imag : ComplexToRealImag
  Delay{,1..7} (8 alike) : Delay  DelayLength=1
  Delay{8..13} (6 alike) : Delay
  Product : Product
  Product1 : Product
  Out1 : Outport
  wires:
  Delay13/1 -> Add/2
  Delay12/1 -> Product1/2
  Delay11/1 -> Product1/1
  Delay10/1 -> Add/1
  Delay9/1 -> Product/2
  Delay8/1 -> Product/1
  Complex to Real-Imag/2 -> Delay4/1, Add2/2
  Delay7/1 -> Add2/1
  Delay4/1 -> Delay5/1
  Delay6/1 -> Delay7/1
  Add2/1 -> Delay12/1
  Delay5/1 -> Delay6/1, Delay11/1
  Delay1/1 -> Delay8/1, Delay2/1
  Add1/1 -> Delay9/1
  Delay2/1 -> Delay3/1
  Delay/1 -> Delay1/1
  Delay3/1 -> Add1/1
  Complex to Real-Imag/1 -> Delay/1, Add1/2
  In1/1 -> Complex to Real-Imag/1
  Add/1 -> Out1/1
  Product1/1 -> Delay13/1
  Product/1 -> Delay10/1

== system commhdlQPSKTxRxLoopback/TxRxComposite/Receiver/QPSK Rx/Frequency and Time Synchronizer/Symbol Synchronizer/No HDL/No HDL ==
  data : Inport
  Enable : EnablePort
  Data Type Conversion : DataTypeConversion  OutDataTypeStr=double  SaturateOnIntegerOverflow=off  RndMeth=Floor
  wires:
  data/1 -> Data Type Conversion/1
  Data Type Conversion/1 -> ?

== system commhdlQPSKTxRxLoopback/TxRxComposite/Receiver/QPSK Rx/Frequency and Time Synchronizer/Symbol Synchronizer/Rate Handle/FIFO ==
  in : Inport
  push : Inport  Port=2
  pop : Inport  Port=3
  reset : Inport  Port=4
  Delay1 : Delay  DelayLength=1
  Pop Counter : hdlsllib/Sources/HDL Counter  CountType=Count limited  CountInit=0  CountStep=1  CountMax=fifoSize -1  CountFromType=Initial value  CountFrom=0  CountResetPort=on  CountLoadPort=off  CountEnbPort=on  CountDirPort=off  CountHitOutputPort=off  CountDataType=Unsigned  CountWordLen=nextpow2(fifoSize)  CountFracLen=0  CountSampTime=1
  Push Counter : hdlsllib/Sources/HDL Counter  CountType=Count limited  CountInit=0  CountStep=1  CountMax=fifoSize -1  CountFromType=Initial value  CountFrom=0  CountResetPort=on  CountLoadPort=off  CountEnbPort=on  CountDirPort=off  CountHitOutputPort=off  CountDataType=Unsigned  CountWordLen=nextpow2(fifoSize)  CountFracLen=0  CountSampTime=1
  Simple Dual Port RAM : hdlsllib/HDL RAMs/Simple Dual Port RAM  ram_size=nextpow2(fifoSize)
  Validate Input Push Pop : Subsystem
  out : Outport
  numEntries : Outport  Port=2
  validPop : Outport  Port=3
  wires:
  Validate Input Push Pop/3(numEntries) -> numEntries/1
  Simple Dual Port RAM/1 -> out/1
  Push Counter/1 -> Simple Dual Port RAM/2
  Pop Counter/1 -> Simple Dual Port RAM/4
  push/1 -> Validate Input Push Pop/2(push)
  pop/1 -> Validate Input Push Pop/3(pop)
  Validate Input Push Pop/1(valid push) -> Simple Dual Port RAM/3, Push Counter/2
  Validate Input Push Pop/2(valid pop) -> validPop/1, Pop Counter/2
  reset/1 -> Delay1/1, Validate Input Push Pop/1(rst)
  in/1 -> Simple Dual Port RAM/1
  Delay1/1 -> Pop Counter/1, Push Counter/1

== system commhdlQPSKTxRxLoopback/TxRxComposite/Transmitter/QPSK Tx/Bit Packetizer/Data Bits FIFO/No HDL/No HDL ==
  push : Inport
  full : Inport  Port=2
  ncount : Inport  Port=3
  empty : Inport  Port=4
  pop : Inport  Port=5
  Assertion : Assertion
  Assertion1 : Assertion
  Display : Display
  Logical Operator : Logic  Operator=NAND  AllPortsSameDT=off  OutDataTypeStr=boolean
  Logical Operator1 : Logic  Operator=NAND  AllPortsSameDT=off  OutDataTypeStr=boolean
  wires:
  push/1 -> Logical Operator/1
  empty/1 -> Logical Operator1/1
  full/1 -> Logical Operator/2
  pop/1 -> Logical Operator1/2
  Logical Operator/1 -> Assertion/1
  ncount/1 -> Display/1
  Logical Operator1/1 -> Assertion1/1

== system commhdlQPSKTxRxLoopback/Receiver/QPSK Rx/Frequency and Time Synchronizer/Symbol Synchronizer/Rate Handle/FIFO/Validate Input Push Pop/No HDL ==
  pushFullFIFO : Inport
  popEmptyFIFO : Inport  Port=2
  Constant2 : Constant  Value=pushFullDiag  SampleTime=-1
  Constant3 : Constant  Value=popEmptyDiag  SampleTime=-1
  MATLAB Function : MATLAB Function  TreatAsAtomicUnit=on
  wires:
  Constant2/1 -> MATLAB Function/1(pushFullDiag)
  Constant3/1 -> MATLAB Function/2(popEmptyDiag)
  popEmptyFIFO/1 -> MATLAB Function/4(popEmpty)
  pushFullFIFO/1 -> MATLAB Function/3(pushFull)

== system commhdlQPSKTxRxLoopback/TxRxComposite/Receiver/QPSK Rx/Frequency and Time Synchronizer/Coarse Frequency Compensator/Coarse Frequency Estimator/Integrator/Reset Generator ==
  validIn : Inport
  Compare To Constant : simulink/Logic and Bit Operations/Compare To Constant  relop===  const=integAvgLen  OutDataTypeStr=boolean
  Delay1 : Delay  DelayLength=1
  Delay5 : Delay  DelayLength=1
  HDL Counter : hdlsllib/Sources/HDL Counter  CountType=Count limited  CountInit=0  CountStep=1  CountMax=integAvgLen  CountFromType=Initial value  CountFrom=0  CountResetPort=off  CountLoadPort=off  CountEnbPort=on  CountDirPort=off  CountHitOutputPort=off  CountDataType=Unsigned  CountWordLen=nextpow2(integAvgLen + 1)  CountFracLen=0  CountSampTime=1
  Logical Operator : Logic  AllPortsSameDT=off  OutDataTypeStr=boolean
  reset : Outport
  wires:
  HDL Counter/1 -> Delay5/1
  Compare To Constant/1 -> Logical Operator/2
  validIn/1 -> Delay1/1, HDL Counter/1
  Logical Operator/1 -> reset/1
  Delay5/1 -> Compare To Constant/1
  Delay1/1 -> Logical Operator/1

== system commhdlQPSKTxRxLoopback/TxRxComposite/Receiver/QPSK Rx/Frequency and Time Synchronizer/Phase Ambiguity Estimation and Correction/Phase Ambiguity Corrector/Reciprocal/Function Impl ==
  switch : Inport
  LUTAddr : Inport  Port=2
  Delay{6..8,10,15..16} (6 alike) : Delay
  Delay9 : Delay  DelayLength=1
  LUT1 : LookupNDDirect  NumberOfTableDimensions=1  Table=LUT(:,1)  DiagnosticForOutOfRangeInput=Error
  LUT2 : LookupNDDirect  NumberOfTableDimensions=1  Table=LUT(:,2)  DiagnosticForOutOfRangeInput=Error
  Multiport Switch : MultiPortSwitch  DataPortOrder=Zero-based contiguous  Inputs=2  zeroidx=on  SaturateOnIntegerOverflow=off  InputSameDT=off
  functionValues : Outport
  wires:
  LUTAddr/1 -> Delay7/1, Delay6/1
  Delay15/1 -> Multiport Switch/2
  Delay16/1 -> Multiport Switch/3
  Delay10/1 -> Multiport Switch/1
  Delay9/1 -> functionValues/1
  LUT2/1 -> Delay15/1
  LUT1/1 -> Delay16/1
  switch/1 -> Delay8/1
  Delay8/1 -> Delay10/1
  Delay7/1 -> LUT2/1
  Delay6/1 -> LUT1/1
  Multiport Switch/1 -> Delay9/1

== system commhdlQPSKTxRxLoopback/TxRxComposite/Receiver/QPSK Rx/Frequency and Time Synchronizer/Preamble Detector/FIFO/Validate Input Push Pop/No HDL ==
  pushFullFIFO : Inport
  popEmptyFIFO : Inport  Port=2
  Constant2 : Constant  Value=pushFullDiag  SampleTime=-1
  Constant3 : Constant  Value=popEmptyDiag  SampleTime=-1
  MATLAB Function : MATLAB Function  TreatAsAtomicUnit=on
  wires:
  pushFullFIFO/1 -> MATLAB Function/3(pushFull)
  popEmptyFIFO/1 -> MATLAB Function/4(popEmpty)
  Constant3/1 -> MATLAB Function/2(popEmptyDiag)
  Constant2/1 -> MATLAB Function/1(pushFullDiag)

== system commhdlQPSKTxRxLoopback/TxRxComposite/Receiver/QPSK Rx/Frequency and Time Synchronizer/Preamble Detector/Timing Adjust/No HDL/No HDL ==
  timingOffset : Inport
  Enable : EnablePort
  Data Type Conversion : DataTypeConversion  OutDataTypeStr=double  SaturateOnIntegerOverflow=off  RndMeth=Floor
  wires:
  timingOffset/1 -> Data Type Conversion/1
  Data Type Conversion/1 -> ?

== system commhdlQPSKTxRxLoopback/TxRxComposite/Receiver/QPSK Rx/Frequency and Time Synchronizer/Preamble Detector/Timing Adjust/No HDL/No HDL1 ==
  frameNumber : Inport
  Enable : EnablePort
  Data Type Conversion : DataTypeConversion  OutDataTypeStr=double  SaturateOnIntegerOverflow=off  RndMeth=Floor
  wires:
  Data Type Conversion/1 -> ?
  frameNumber/1 -> Data Type Conversion/1

== system commhdlQPSKTxRxLoopback/TxRxComposite/Receiver/QPSK Rx/Frequency and Time Synchronizer/Symbol Synchronizer/Rate Handle/FIFO/Validate Input Push Pop ==
  rst : Inport
  push : Inport  Port=2
  pop : Inport  Port=3
  Compare To Constant : hdlsllib/Logic and Bit Operations/Compare To Constant  relop===  const=0  OutDataTypeStr=boolean
  Compare To Constant1 : hdlsllib/Logic and Bit Operations/Compare To Constant  relop===  const=fifoSize  OutDataTypeStr=boolean
  Constant : Constant  Value=true  SampleTime=-1
  Constant1 : Constant  Value=false  SampleTime=-1
  Delay : Delay  DelayLength=1
  Logical Operator1 : Logic  Operator=XOR  AllPortsSameDT=off  OutDataTypeStr=boolean
  Logical Operator2 : Logic  Operator=NOT  AllPortsSameDT=off  OutDataTypeStr=boolean
  Logical Operator{3..5,7,9} (5 alike) : Logic  AllPortsSameDT=off  OutDataTypeStr=boolean
  Logical Operator6 : Logic  Operator=NOT  AllPortsSameDT=off  OutDataTypeStr=boolean
  Logical Operator8 : Logic  Operator=NOT  AllPortsSameDT=off  OutDataTypeStr=boolean
  MATLAB Function : MATLAB Function  TreatAsAtomicUnit=on  mask{initVal=0, countToVal=fifoSize}
      mask prompts: initVal "Initial value:"; countToVal "Count to value:"
  No HDL : Subsystem
  Switch : Switch  Criteria=u2 ~= 0  SaturateOnIntegerOverflow=off  InputSameDT=off
  valid push : Outport
  valid pop : Outport  Port=2
  numEntries : Outport  Port=3
  wires:
  Delay/1 -> Compare To Constant/1, numEntries/1, Compare To Constant1/1
  rst/1 -> MATLAB Function/1(rst)
  Compare To Constant/1 -> Logical Operator3/1
  pop/1 -> Logical Operator7/1, Logical Operator3/2
  Switch/1 -> MATLAB Function/3(dir)
  MATLAB Function/1(count) -> Delay/1
  Constant1/1 -> Switch/1
  Logical Operator3/1 -> Logical Operator6/1, No HDL/2(popEmptyFIFO)  "pop on empty FIFO"
  Logical Operator4/1 -> Logical Operator2/1, No HDL/1(pushFullFIFO)  "push on full FIFO"
  Constant/1 -> Switch/3
  Compare To Constant1/1 -> Logical Operator4/2
  Logical Operator7/1 -> Logical Operator1/2, Logical Operator8/1, valid pop/1, Switch/2
  Logical Operator6/1 -> Logical Operator7/2
  Logical Operator1/1 -> MATLAB Function/2(enb)
  push/1 -> Logical Operator9/1, Logical Operator5/1
  Logical Operator8/1 -> Logical Operator5/2
  Logical Operator5/1 -> Logical Operator4/1
  Logical Operator2/1 -> Logical Operator9/2
  Logical Operator9/1 -> valid push/1, Logical Operator1/1

== system commhdlQPSKTxRxLoopback/TxRxComposite/Receiver/QPSK Rx/Frequency and Time Synchronizer/Symbol Synchronizer/Rate Handle/FIFO/Validate Input Push Pop/No HDL ==
  pushFullFIFO : Inport
  popEmptyFIFO : Inport  Port=2
  Constant2 : Constant  Value=pushFullDiag  SampleTime=-1
  Constant3 : Constant  Value=popEmptyDiag  SampleTime=-1
  MATLAB Function : MATLAB Function  TreatAsAtomicUnit=on
  wires:
  pushFullFIFO/1 -> MATLAB Function/3(pushFull)
  popEmptyFIFO/1 -> MATLAB Function/4(popEmpty)
  Constant3/1 -> MATLAB Function/2(popEmptyDiag)
  Constant2/1 -> MATLAB Function/1(pushFullDiag)

== matlab function commhdlQPSKTxRxLoopback/Receiver/QPSK Rx/Frequency and Time Synchronizer/Symbol Synchronizer/Rate Handle/FIFO/Validate Input Push Pop/No HDL/MATLAB Function ==
  data: pushFullDiag input; popEmptyDiag input; pushFull input; popEmpty input
function pushPopDiagnostics(pushFullDiag, popEmptyDiag, pushFull, popEmpty)
%#codegen


if(pushFull)
    switch pushFullDiag
        case 2
            warning('Push signal applied on full FIFO');
        case 3
            error('Push signal applied on full FIFO');
        otherwise
    end
end

if(popEmpty)
    switch popEmptyDiag
        case 2
            warning('Pop signal applied on empty FIFO');
        case 3
            error('Pop signal applied on empty FIFO');
        otherwise
    end
end

end

== matlab function commhdlQPSKTxRxLoopback/Receiver/Capture Data Bits/MATLAB Function ==
  data: valid input; datain input; start input; stop input; count_out output; packets_out output; bit_errors_out output
function [count_out, packets_out, bit_errors_out] = msgdec(valid, datain, start, stop)

persistent count;
persistent msgbuffer;

persistent packetsReceived
persistent errors;

if isempty(count) || isempty(msgbuffer) || isempty(packetsReceived)
    count = uint32(0);
    msgbuffer = zeros(1,120+8)>0; % ADI Hello WorldX
    packetsReceived = uint32(0);
    errors = uint32(0);
end

% Mesg
strAscii = dec2bin('ADI Hello World',8);
msgarray = reshape(strAscii', [1, numel(strAscii)]);
msgbits = logical(msgarray - 48);

% msgLen = uint32(2240);

if valid
    if start
        count = uint32(1);
        packetsReceived = packetsReceived + 1;
    end

    if count <= (length(msgbuffer) - 8)
        msgbuffer(count) = datain;
        if datain ~= msgbits(count)
            errors = errors + 1;
        end

    elseif count == length(msgbuffer) + 1
        msgarray_dec = char('0' + msgbuffer);
        N = length(msgarray_dec) / 8;
        strAscii_dec = reshape(msgarray_dec , 8, N).';
        msg = char(bin2dec(strAscii_dec).');
        disp(msg);
    end
    
    if count <= length(msgbuffer) + 2
        count = count + 1;
    end
end

count_out = count;
packets_out = packetsReceived;
bit_errors_out = errors;
